simulink model "pendulum"  (R2024b)
settings: Solver=ode4  StartTime=0.0  StopTime=10  FixedStep=0.01  RelTol=1e-3
model workspace (MAT data in the model file):
  I = 0.0007176
  M = 0.136
  b = 7.892e-05
  c = 0.63
  g = 9.81
  l = 0.2
  m = 0.1
  theta0 = 0.1
  u_force = 0
  x0 = 0
Description:
  | Pendule inverse sur chariot. Derive de IP_Nonlinear_model.slx de Jitendra Singh (MIT, https://github.com/jitendra825/Inverted-Pendulum-Simulink). Voir LICENSE-modele.txt et build_cartpole_simulink.m.
settings Model: Creator=jitendra  LastModifiedBy=krist
settings SolverCC: AlgebraicLoopSolver=TrustRegion
settings DataIOCC: ExternalInput=getinputstruct(op_trim1)  InitialState=getstatestruct(op_trim1)  ReturnWorkspaceOutputs=off
settings DebuggingCC: AlgebraicLoopMsg=none  UnconnectedInputMsg=warning  UnconnectedOutputMsg=warning  UnconnectedLineMsg=warning  ArithmeticOperatorsInVariantConditions=warning
settings ModelReferenceCC: EnableRefExpFcnMdlSchedulingChecks=on
settings SFSimCC: SimUseLocalCustomCode=off  CustomCodeUndefinedFunction=UseInterfaceOnly
settings RTWCC: RTWUseLocalCustomCode=off  GPUComputeCapability=3.5
settings ConfigComp: CovMetricSettings=de  CovBoundaryAbsTol=1.0e-5

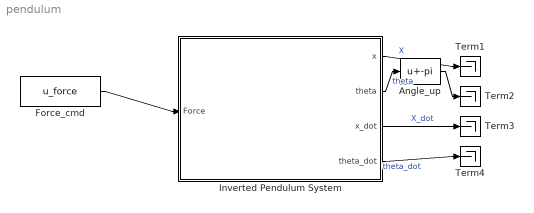
== system pendulum ==
  Angle_up : Bias  Bias=-pi  SaturateOnIntegerOverflow=off
  Force_cmd : Constant  Value=u_force
  Inverted Pendulum System : Subsystem
      mask Display: image('ip_model.png');
  Term{1..4} (4 alike) : Terminator
  wires:
  Force_cmd/1 -> Inverted Pendulum System/1(Force)
  Inverted Pendulum System/1(x) -> Term1/1  "X"
  Inverted Pendulum System/2(theta) -> Angle_up/1  "theta"
  Angle_up/1 -> Term2/1
  Inverted Pendulum System/3(x_dot) -> Term3/1  "X_dot"
  Inverted Pendulum System/4(theta_dot) -> Term4/1  "theta_dot"

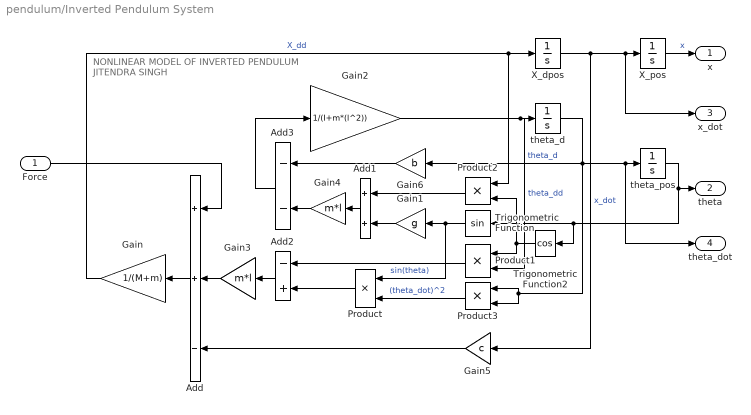
== system pendulum/Inverted Pendulum System ==
  note: NONLINEAR MODEL OF
      | INVERTED PENDULUM
      | JITENDRA SINGH
  Force : Inport
  Add : Sum  Inputs=++-
  Add1 : Sum
  Add2 : Sum  Inputs=-+
  Add3 : Sum  Inputs=--
  Gain : Gain  Gain=1/(M+m)
  Gain1 : Gain  Gain=g
  Gain2 : Gain  Gain=1/(I+m*(l^2))
  Gain3 : Gain  Gain=m*l
  Gain4 : Gain  Gain=m*l
  Gain5 : Gain  Gain=c
  Gain6 : Gain  Gain=b
  Product{,1..3} (4 alike) : Product
  Trigonometric Function : Trigonometry
  Trigonometric Function2 : Trigonometry  Operator=cos
  X_dpos : Integrator
  X_pos : Integrator  InitialCondition=x0
  theta_d : Integrator
  theta_pos : Integrator  InitialCondition=pi + theta0
  x : Outport  VectorParamsAs1DForOutWhenUnconnected=off
  theta : Outport  Port=2  VectorParamsAs1DForOutWhenUnconnected=off
  x_dot : Outport  Port=3  VectorParamsAs1DForOutWhenUnconnected=off
  theta_dot : Outport  Port=4  VectorParamsAs1DForOutWhenUnconnected=off
  wires:
  Gain5/1 -> Add/3
  Add2/1 -> Gain3/1
  Add3/1 -> Gain2/1
  Trigonometric Function2/1 -> Product2/2, Product1/1
  Trigonometric Function/1 -> Product/1, Gain1/1  "sin(theta)"
  Gain3/1 -> Add/2
  theta_d/1 -> Product3/2, Product3/1, Gain6/1, theta_dot/1, theta_pos/1  "theta_d"
  Product2/1 -> Add1/1
  Product/1 -> Add2/2
  Gain4/1 -> Add3/2
  Product3/1 -> Product/2  "(theta_dot)^2"
  X_pos/1 -> x/1  "x"
  Product1/1 -> Add2/1
  Gain/1 -> X_dpos/1, Product2/1  "X_dd"
  Add/1 -> Gain/1
  Gain2/1 -> Product1/2, theta_d/1  "theta_dd"
  Gain6/1 -> Add3/1
  theta_pos/1 -> Trigonometric Function2/1, Trigonometric Function/1, theta/1
  Force/1 -> Add/1
  Gain1/1 -> Add1/2
  X_dpos/1 -> x_dot/1, X_pos/1, Gain5/1  "x_dot"
  Add1/1 -> Gain4/1
